simulink library "PID_costum"  (R2022b)
settings: Solver=VariableStepAuto  StartTime=0.0  StopTime=10.0  RelTol=1e-3
libraries: simulink x1
settings Model: Creator=asoltanieh  LastModifiedBy=asoltanieh

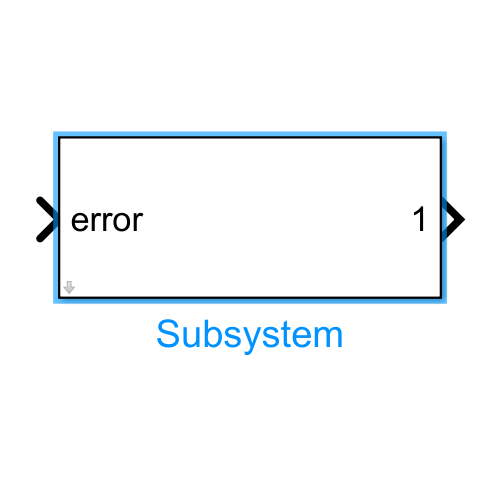
[thumbnail: Simulink's stored preview of the top-level diagram]
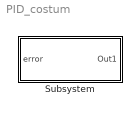
== system PID_costum ==
  Subsystem : Subsystem  mask{K_P=0, K_I=0, K_D=0, Sat_value=0.01}
      mask prompts: K_P "kp"; K_I "ki"; K_D "kd"; Sat_value "Saturation Value"

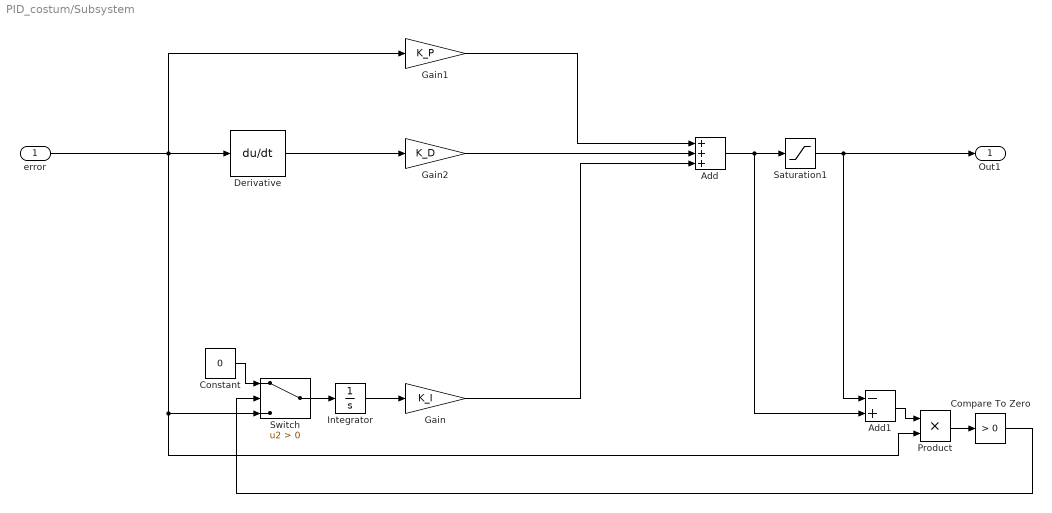
== system PID_costum/Subsystem ==
  error : Inport
  Add : Sum  Inputs=+++
  Add1 : Sum  Inputs=-+
  Compare To Zero : simulink/Logic and Bit Operations/Compare To Zero  relop=>  OutDataTypeStr=boolean
  Constant : Constant  Value=0
  Derivative : Derivative
  Gain : Gain  Gain=K_I
  Gain1 : Gain  Gain=K_P
  Gain2 : Gain  Gain=K_D
  Integrator : Integrator
  Product : Product
  Saturation1 : Saturate  UpperLimit=Sat_value  LowerLimit=-Sat_value
  Switch : Switch  Criteria=u2 > Threshold  SaturateOnIntegerOverflow=off  InputSameDT=off
  Out1 : Outport
  wires:
  Gain1/1 -> Add/1
  Integrator/1 -> Gain/1
  Add/1 -> Add1/2, Saturation1/1
  Derivative/1 -> Gain2/1
  Gain2/1 -> Add/2
  Add1/1 -> Product/1
  Compare To Zero/1 -> Switch/2
  Constant/1 -> Switch/1
  Saturation1/1 -> Add1/1, Out1/1
  Switch/1 -> Integrator/1
  error/1 -> Product/2, Switch/3, Derivative/1, Gain1/1
  Gain/1 -> Add/3
  Product/1 -> Compare To Zero/1
